simulink model "throttle_valve_simulink"  (R2026a)
settings: Solver=ode3  FixedStep=.001
libraries: simulink x3, slpidlib x2
settings Model: Creator=Noah  LastModifiedBy=asing
settings SFSimCC: SimGPUStackLimitPerThread=51200
settings RTWCC: GPUStackLimitPerThread=51200

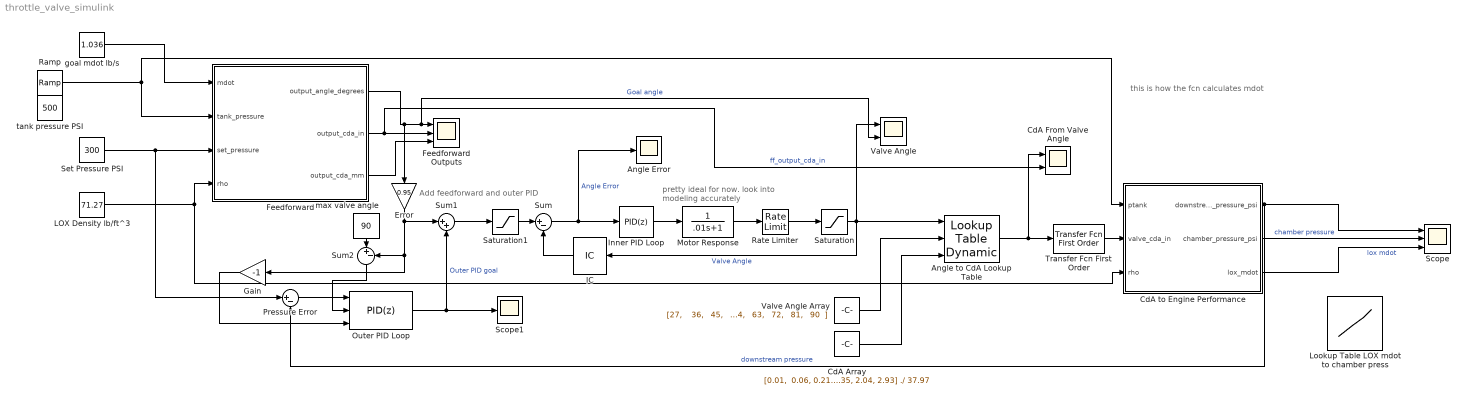
== system throttle_valve_simulink ==
  note: Add feedforward and outer PID
  note: pretty ideal for now. look into modeling accurately
  note: this is how the fcn calculates mdot
  Angle Error : Scope
      settings: ActiveDisplayYMinimum=-1.9778402233924819  ActiveDisplayYMaximum=97.477324384222584  DataLoggingVariableName=ScopeData2
  Angle to CdA Lookup Table : simulink/Lookup Tables/Lookup Table Dynamic  LookUpMeth=Interpolation-Use End Values  OutDataType=fixdt('double')  OutScaling=[]  OutputDataTypeScalingMode=Specify via dialog  OutDataTypeStr=double  DoSatur=off
  CdA Array : Constant  Value="[0.01,  0.06, 0.21, 0.46, 0.83, 1.35, 2.04, 2.93] ./ 37.97"
  CdA From Valve Angle : Scope  NumInputPorts=2
      settings: ActiveDisplayYMinimum=-0.011018908191937576  ActiveDisplayYMaximum=0.025312171715467451  DataLoggingVariableName=ScopeData3
  CdA to Engine Performance : MATLAB Function  TreatAsAtomicUnit=on
  Error : Gain  Gain=0.95
  Feedforward : MATLAB Function  TreatAsAtomicUnit=on
  Feedforward Outputs : Scope  NumInputPorts=3
      settings: ActiveDisplayYMinimum=16.254870819281589  ActiveDisplayYMaximum=58.754487056953195
  Gain : Gain  Gain=-1
  IC : InitialCondition  Value=0
  Inner PID Loop : slpidlib/PID Controller  Controller=PID  Form=Parallel  TimeDomain=Discrete-time  UseExternalTs=off  SampleTime=0.001  IntegratorMethod=Forward Euler  FilterMethod=Forward Euler  ControllerParametersSource=internal  P=0.2  I=20  UseKiTs=off  D=0  UseExternalDerivativeSource=off  N=100  UseFilter=on  TunerSelectOption=Transfer Function Based (PID Tuner App)  InitialConditionSource=internal  InitialConditionForIntegrator=0  InitialConditionForFilter=0  DifferentiatorICPrevScaledInput=0  ExternalReset=none  TrackingMode=off  Kt=1  LimitOutput=on  SatLimitsSource=internal  UpperSaturationLimit=90  LowerSaturationLimit=0  LinearizeAsGain=off  AntiWindupMode=clamping  Kb=1  LimitIntegrator=off  UpperIntegratorSaturationLimit=inf  LowerIntegratorSaturationLimit=-inf  POutMin=[]  POutMax=[]  IOutMin=[]  IOutMax=[]  DOutMin=[]  DOutMax=[]  NOutMin=[]  NOutMax=[]  SumOutMin=[]  SumOutMax=[]  SaturationOutMin=[]  SaturationOutMax=[]  PParamMin=[]  PParamMax=[]  IParamMin=[]  IParamMax=[]  DParamMin=[]  DParamMax=[]  NParamMin=[]  NParamMax=[]  KbParamMin=[]  KbParamMax=[]  KtParamMin=[]  KtParamMax=[]  KbOutMin=[]  KbOutMax=[]  KtOutMin=[]  KtOutMax=[]  IntegratorOutMin=[]  IntegratorOutMax=[]  FilterOutMin=[]  FilterOutMax=[]  SumI1OutMin=[]  SumI1OutMax=[]  SumI2OutMin=[]  SumI2OutMax=[]  SumI3OutMin=[]  SumI3OutMax=[]  SumI4OutMin=[]  SumI4OutMax=[]  SumDOutMin=[]  SumDOutMax=[]  DifferentiatorOutMin=[]  DifferentiatorOutMax=[]  FilterDiffOutCoefMin=[]  FilterDiffOutCoefMax=[]  ReciprocalOutMin=[]  ReciprocalOutMax=[]  SumDenOutMin=[]  SumDenOutMax=[]  SumNumOutMin=[]  SumNumOutMax=[]  DivideOutMin=[]  DivideOutMax=[]  UdiffTsProdOutMin=[]  UdiffTsProdOutMax=[]  NTsProdOutMin=[]  NTsProdOutMax=[]  UintegralTsProdOutMin=[]  UintegralTsProdOutMax=[]  UngainTsProdOutMin=[]  UngainTsProdOutMax=[]  ClampingZeroOutDataTypeStr=Inherit: Inherit via back propagation  ClampingZeroOutMin=[]  ClampingZeroOutMax=[]  FilterDenConstantOutDataTypeStr=Inherit: Inherit via back propagation  FilterDenConstantOutMin=[]  FilterDenConstantOutMax=[]  PCopyOutDataTypeStr=Inherit: Inherit via back propagation  PCopyOutMin=[]  PCopyOutMax=[]  NCopyOutDataTypeStr=Inherit: Inherit via back propagation  NCopyOutMin=[]  NCopyOutMax=[]  IntegratorContinuousStateAttributes=''  IntegratorStateMustResolveToSignalObject=off  IntegratorRTWStateStorageClass=Auto  FilterContinuousStateAttributes=''  FilterStateMustResolveToSignalObject=off  FilterRTWStateStorageClass=Auto  ParallelPVariant=InternalParameters  IdealPVariant=Disabled  IVariant=InternalParameters  DVariant=InternalParameters  IntegratorVariant=Discrete  SatVariant=Enabled  AWVariant=DiscClampingParallel  PCopyVariant=Disabled  TRVariant=Disabled  FdbkBlocksVariant=Forward  IdealPFdbkVariant=Disabled  SatFdbkVariant=Disabled  DerivativeFilterVariant=ForwardEulerFilter  NVariant=InternalParameters  NCopyVariant=Disabled  FilterICVariant=InternalICsFilter  IntegratorICVariant=InternalICs  ExternalResetVariant=Disabled  TRSumVariant=Passthrough  SumFdbkVariant=Disabled  SumVariant=Sum_PID  TsampFilterVariant=InternalTs  TsampNgainVariant=Passthrough  TsampIntegralVariant=Disabled_SignalSpec  ExternalSaturationOutDataTypeStr=Inherit: Same as second input  DerivativeSourceVariant=ErrorSignal  PreIntVariant=InternalPreInt
      settings: LibrarySourceBlock=simulink/Discrete/Discrete PID Controller
  LOX Density lb/ft^3 : Constant  Value=71.27
  Lookup Table LOX mdot to chamber press : Lookup_n-D  NumberOfTableDimensions=1  BreakpointsForDimension1=[0.3256, 0.3331, 0.3432, 0.3582, 0.3809, 0.406, 0.4311, 0.4563, 0.4814, 0.5063, 0.5302, 0.5541, 0.5778, 0.6014]  Table=[144.02, 160.72, 169.84, 178.25, 189.59, 202.13, 214.7, 227.27, 239.84, 252.3, 264.31, 276.25, 288.13, 299.74]  InternalRulePriority=Speed  RndMeth=Simplest
  Motor Response : TransferFcn  Denominator=[.01 1]  ContinuousStateAttributes='position'
  Outer PID Loop : slpidlib/PID Controller  Controller=PID  Form=Parallel  TimeDomain=Discrete-time  UseExternalTs=off  SampleTime=0.005  IntegratorMethod=Forward Euler  FilterMethod=Forward Euler  ControllerParametersSource=internal  P=0.085  I=0.2  UseKiTs=off  D=0  UseExternalDerivativeSource=off  N=100  UseFilter=on  TunerSelectOption=Transfer Function Based (PID Tuner App)  InitialConditionSource=internal  InitialConditionForIntegrator=0  InitialConditionForFilter=0  DifferentiatorICPrevScaledInput=0  ExternalReset=none  TrackingMode=off  Kt=1  LimitOutput=on  SatLimitsSource=external  UpperSaturationLimit=inf  LowerSaturationLimit=-inf  LinearizeAsGain=off  AntiWindupMode=clamping  Kb=1  LimitIntegrator=off  UpperIntegratorSaturationLimit=inf  LowerIntegratorSaturationLimit=-inf  POutMin=[]  POutMax=[]  IOutMin=[]  IOutMax=[]  DOutMin=[]  DOutMax=[]  NOutMin=[]  NOutMax=[]  SumOutMin=[]  SumOutMax=[]  SaturationOutMin=[]  SaturationOutMax=[]  PParamMin=[]  PParamMax=[]  IParamMin=[]  IParamMax=[]  DParamMin=[]  DParamMax=[]  NParamMin=[]  NParamMax=[]  KbParamMin=[]  KbParamMax=[]  KtParamMin=[]  KtParamMax=[]  KbOutMin=[]  KbOutMax=[]  KtOutMin=[]  KtOutMax=[]  IntegratorOutMin=[]  IntegratorOutMax=[]  FilterOutMin=[]  FilterOutMax=[]  SumI1OutMin=[]  SumI1OutMax=[]  SumI2OutMin=[]  SumI2OutMax=[]  SumI3OutMin=[]  SumI3OutMax=[]  SumI4OutMin=[]  SumI4OutMax=[]  SumDOutMin=[]  SumDOutMax=[]  DifferentiatorOutMin=[]  DifferentiatorOutMax=[]  FilterDiffOutCoefMin=[]  FilterDiffOutCoefMax=[]  ReciprocalOutMin=[]  ReciprocalOutMax=[]  SumDenOutMin=[]  SumDenOutMax=[]  SumNumOutMin=[]  SumNumOutMax=[]  DivideOutMin=[]  DivideOutMax=[]  UdiffTsProdOutMin=[]  UdiffTsProdOutMax=[]  NTsProdOutMin=[]  NTsProdOutMax=[]  UintegralTsProdOutMin=[]  UintegralTsProdOutMax=[]  UngainTsProdOutMin=[]  UngainTsProdOutMax=[]  ClampingZeroOutDataTypeStr=Inherit: Inherit via back propagation  ClampingZeroOutMin=[]  ClampingZeroOutMax=[]  FilterDenConstantOutDataTypeStr=Inherit: Inherit via back propagation  FilterDenConstantOutMin=[]  FilterDenConstantOutMax=[]  PCopyOutDataTypeStr=Inherit: Inherit via back propagation  PCopyOutMin=[]  PCopyOutMax=[]  NCopyOutDataTypeStr=Inherit: Inherit via back propagation  NCopyOutMin=[]  NCopyOutMax=[]  IntegratorContinuousStateAttributes=''  IntegratorStateMustResolveToSignalObject=off  IntegratorRTWStateStorageClass=Auto  FilterContinuousStateAttributes=''  FilterStateMustResolveToSignalObject=off  FilterRTWStateStorageClass=Auto  ParallelPVariant=InternalParameters  IdealPVariant=Disabled  IVariant=InternalParameters  DVariant=InternalParameters  IntegratorVariant=Discrete  SatVariant=External  AWVariant=DiscClampingParallel  PCopyVariant=Disabled  TRVariant=Disabled  FdbkBlocksVariant=Forward  IdealPFdbkVariant=Disabled  SatFdbkVariant=Disabled  DerivativeFilterVariant=ForwardEulerFilter  NVariant=InternalParameters  NCopyVariant=Disabled  FilterICVariant=InternalICsFilter  IntegratorICVariant=InternalICs  ExternalResetVariant=Disabled  TRSumVariant=Passthrough  SumFdbkVariant=Disabled  SumVariant=Sum_PID  TsampFilterVariant=InternalTs  TsampNgainVariant=Passthrough  TsampIntegralVariant=Disabled_SignalSpec  ExternalSaturationOutDataTypeStr=Inherit: Same as second input  DerivativeSourceVariant=ErrorSignal  PreIntVariant=InternalPreInt
      settings: LibrarySourceBlock=simulink/Discrete/Discrete PID Controller
  Pressure Error : Sum  Inputs=|+-
  Ramp : simulink/Sources/Ramp  slope=-5  start=0  InitialOutput=500
  Rate Limiter : RateLimiter  RisingSlewLimit=2062  FallingSlewLimit=-2062  SampleTimeMode=inherited
  Saturation : Saturate  UpperLimit=90  LowerLimit=0
  Saturation1 : Saturate  UpperLimit=90  LowerLimit=0
  Scope : Scope  NumInputPorts=3
      settings: ActiveDisplayYMinimum=-37.104058003728532  ActiveDisplayYMaximum=341.45827599811355  DataLoggingVariableName=ScopeData4
  Scope1 : Scope
      settings: ActiveDisplayYMinimum=-28.527076555530527  ActiveDisplayYMaximum=141.3243379131022  DataLoggingVariableName=ScopeData5
  Set Pressure PSI : Constant  Value=300
  Sum : Sum  Inputs=|+-
  Sum1 : Sum  Inputs=|++
  Sum2 : Sum  Inputs=|+-
  Transfer Fcn First Order : simulink/Discrete/Transfer Fcn First Order  PoleZ=0.9  ICPrevOutput=0.0  DoSatur=off
  Valve Angle : Scope  NumInputPorts=2
      settings: ActiveDisplayYMinimum=36.979156056338425  ActiveDisplayYMaximum=63.942012098069952
  Valve Angle Array : Constant  Value="[27,    36,   45,   54,   63,   72,   81,   90  ]"
  goal mdot lb/s : Constant  Value=1.036
  max valve angle : Constant  Value=90
  tank pressure PSI : Constant  Value=500
  wires:
  goal mdot lb/s/1 -> Feedforward/1(mdot)
  Ramp/1 -> Feedforward/2(tank_pressure), CdA to Engine Performance/1(ptank)
  Set Pressure PSI/1 -> Pressure Error/1, Feedforward/3(set_pressure)
  LOX Density lb/ft^3/1 -> CdA to Engine Performance/3(rho), Feedforward/4(rho)
  Feedforward/1(output_angle_degrees) -> Error/1, Feedforward Outputs/1, Valve Angle/2  "Goal angle"
  Feedforward/2(output_cda_in) -> Feedforward Outputs/2, CdA From Valve Angle/2  "ff_output_cda_in"
  Feedforward/3(output_cda_mm) -> Feedforward Outputs/3
  Sum/1 -> Inner PID Loop/1, Angle Error/1  "Angle Error"
  Inner PID Loop/1 -> Motor Response/1
  Motor Response/1 -> Rate Limiter/1
  Saturation/1 -> Angle to CdA Lookup Table/1, Valve Angle/1, IC/1  "Valve Angle"
  Rate Limiter/1 -> Saturation/1
  IC/1 -> Sum/2
  CdA Array/1 -> Angle to CdA Lookup Table/3
  Valve Angle Array/1 -> Angle to CdA Lookup Table/2
  Angle to CdA Lookup Table/1 -> CdA From Valve Angle/1, Transfer Fcn First Order/1
  CdA to Engine Performance/2(chamber_pressure_psi) -> Scope/2  "chamber pressure"
  CdA to Engine Performance/1(downstream_pressure_psi) -> Pressure Error/2, Scope/1  "downstream pressure"
  CdA to Engine Performance/3(lox_mdot) -> Scope/3  "lox mdot"
  Transfer Fcn First Order/1 -> CdA to Engine Performance/2(valve_cda_in)
  Pressure Error/1 -> Outer PID Loop/1
  Sum1/1 -> Saturation1/1
  Outer PID Loop/1 -> Scope1/1, Sum1/2  "Outer PID goal"
  Saturation1/1 -> Sum/1
  Error/1 -> Sum2/2, Gain/1, Sum1/1
  Gain/1 -> Outer PID Loop/3
  Sum2/1 -> Outer PID Loop/2
  max valve angle/1 -> Sum2/1

== matlab function throttle_valve_simulink/CdA to Engine Performance ==
  data: ptank input; valve_cda_in input; rho input; downstream_pressure_psi output; chamber_pressure_psi output; lox_mdot output
% calculates chamber pressure, downstream pressure, and lox mdot based on
% valve angle and upstream pressure
function [downstream_pressure_psi, chamber_pressure_psi, lox_mdot] = fcn(ptank, valve_cda_in, rho)
%all units m, Pa, kg. convert to imperial at end

k = 3.44e6; % uses Pc = mdot * cstar / At. will get dynamic calculation later but this is an approximation for now
injector_cda_m = 15.3e-6;

rho = rho * 16.01846337; % lb/ft^3 to kg/m^3
ptank = ptank * 6894.75729; % psi to pa
valve_cda_m = valve_cda_in * 0.00064516; %convert in^2 to m^2

a = (1/valve_cda_m^2 + 1/injector_cda_m^2)/(2 * rho);

lox_mdot = 2*ptank/(k + sqrt(k^2 + 4*a*ptank));
chamber_pressure_pa = k * lox_mdot;
downstream_pressure_pa = chamber_pressure_pa + lox_mdot^2/(2 * rho * injector_cda_m^2);


chamber_pressure_psi = chamber_pressure_pa * 0.000145038;
downstream_pressure_psi = downstream_pressure_pa * 0.000145038;

== matlab function throttle_valve_simulink/Feedforward ==
  data: mdot input; tank_pressure input; set_pressure input; rho input; output_angle_degrees output; output_cda_in output; output_cda_mm output
%takes in goal mass flow rate and downstream pressure, uses density and
%tank upstream(tank) pressure to predict the valve angle using a lookup
%table
function [output_angle_degrees, output_cda_in, output_cda_mm] = fcn(mdot, tank_pressure, set_pressure, rho)
    gc = 32.174;

    dp = max(tank_pressure - set_pressure, 1e-6); % divide by zero error

    dp_lb_ft = dp * 144;
    % calculate CdA in ft^2, then convert to in^2
    output_cda_in = 144 * (mdot / sqrt(2 * dp_lb_ft * rho * gc));
    
    output_cda_in = max(output_cda_in, 1e-7); % divide by zero error
    output_cda_mm = output_cda_in * 645.16;

    %Cv vector divided by 37.97
    cda_vector =   [0.01,  0.06, 0.21, 0.46, 0.83, 1.35, 2.04, 2.93] ./ 37.97;
    theta_vector = [27,    36,   45,   54,   63,   72,   81,   90  ]; % 9 degree increments
    
    output_angle_degrees = interp1(cda_vector, theta_vector, output_cda_in);
    output_angle_degrees = min(output_angle_degrees, 90);
    output_angle_degrees = max(output_angle_degrees, 0);
